simulink model "ASM_Traffic_new"  (R2024a)
settings: Solver=ode1  StartTime=SIM.tstart.v  StopTime=SIM.tend.v  FixedStep=SIM.StepSize.v  RelTol=1e-3
PostLoadFcn:
  | if any(exist('dsrtsu_mdlpostloadfcn', 'file') ~= 0), dsrtsu_mdlpostloadfcn('Execute', bdroot); end
  | try, asm_mdl_postloadfcn(bdroot, 'UpdateModel', 3600); catch, disp(lasterr); end,
InitFcn:
  | , if any(exist('rtifpga_mdlclblib', 'file') ~= 0), rtifpga_mdlclblib('Init', bdroot); end,
  | , if any(exist('dsmpb_private', 'file') ~= 0), dsmpb_private('dsmpb_mdlclblib', 'Init', bdroot); end,
undefined symbols (not defined in the file): _to_, a0b2, ASM_BrakeHydraulics_DemoSystems, ASM_VehicleDynamics_DemoSystems, b98103fe8ad365046cd0, BrakeCircuit, CPT, Crankshaft, DiscIntNeverNeededParam, dsmsi, FinalDriveAssembly, MDL, ModeSignals, Pos_BrakePedal_Maneuver, rad, RefSignals, s_to_rpm, SIM, SoftECU, Suspension, Tire, Transmission
libraries: ASM_Traffic_lib x135, simulink x100, ASM_Utils_lib x77, ASM_VehicleDynamics_lib x70, ASM_Environment_lib x22, dsmpblib x20, dsmsilib x15, MDLD_Utils_lib x10, ASM_BrakeHydraulics_lib x3
(part 2 of 63)

== system ASM_Traffic_new/ASMTools ==
  note: ---- Code Generation ----
  note: ------ Multi-Instance ------
  note: ----- Scope Handling ------
  note: ----- Signal Handling ------
  note: ------------------- Project & Experiment Handling -------------------
  note: -------------------- ModelDesk Parameter Group --------------------
  note: ------------------------------- Tire Handling -------------------------------
  ASMSignalInterface_Manager : MDLD_Utils_lib/ModelDeskPlotInterface/ASMSignalInterface_Manager
  ASM_Model_Port_Manager : ASM_Utils_lib/Miscellaneous/ASM_MODEL_PORT_MANAGER
  GenerateVEOS : ASM_Utils_lib/CodeGeneration/GenerateVEOS
  ModelDeskParaGroupOverview : ASM_Utils_lib/ModelDeskInterface/ModelDeskParaGroupOverview
  MultiInstanceOverview : ASM_Utils_lib/ModelDeskInterface/MultiInstanceOverview
  OpenExperimentModelDesk : ASM_Utils_lib/OpenExperiment/OpenExperiment  ExpDir=..\Parameterization\MOD_Traffic\Experiment_001\Experiment_001.CDE  dSProduct=ModelDesk
  ReplaceTire : ASM_Utils_lib/BlockReplacement/ReplaceVariants  editSearchPath=bdroot  popupLibBlk=<select here>  popupTargetDemo=<select here>  Demosystem=VehicleDynamics_Tire  variantLib=ASM_VehicleDynamics_DemoSystems/Tire
  ScopeHandlingGui : ASM_Utils_lib/ReplaceScopes/ScopeHandlingGui

== system ASM_Traffic_new/AnimationInterface ==
  note: Animation Interface
  In : Inport
  ANIMATION_INTERFACE : Subsystem
  Bus Selector : BusSelector  OutputSignals=Environment.Animation.Sw_AnimationInterface[0Disabled|1Enabled],Environment.Animation.ManeuverState[]
  DriverAssistance_Animation : BusSelector  OutputSignals=DomainControl.DriverAssistance.Animation  OutputAsBus=on
  Drivetrain_Animation : BusSelector  OutputSignals=Drivetrain.Animation  OutputAsBus=on
  Environment_Animation : BusSelector  OutputSignals=Environment.Animation  OutputAsBus=on
  FcnCall : Subsystem
  Fellow_Doors : Subsystem
  Fellow_Lights : Subsystem
  OpenAnimationInterfaceModel : Subsystem
      settings: OpenFcn=|
      | InterfaceModel = 'ASM_AnimationInterface';
      | 
      | try
      |     open_system(InterfaceModel);                         catch
      |     errordlg(['ERROR opening Animation interface: ',InterfaceModel,'.slx']);
      | end
      mask Display: disp('Open ASM_AnimationInterface')
  Rate Transition{,1..3} (4 alike) : RateTransition  Integrity=off  OutPortSampleTimeOpt=Inherit
  VehicleDynamics_Animation : BusSelector  OutputSignals=VehicleDynamics.Animation  OutputAsBus=on
  Vehicle_Doors : Subsystem
  Vehicle_Lights : Subsystem
  wires:
  Bus Selector/1 -> FcnCall/Enable  "<Sw_AnimationInterface[0Disabled|1Enabled]>"
  Fellow_Doors/1(Fellow_Doors) -> ANIMATION_INTERFACE/8(Fellow_Doors)
  Vehicle_Doors/1(ASM_Vehicle_Doors) -> ANIMATION_INTERFACE/7(ASM_Vehicle_Doors)
  Rate Transition2/1 -> ANIMATION_INTERFACE/4(Environment_Animation), Vehicle_Lights/2(Environment_Animation), Fellow_Doors/1(Environment_Animation), Vehicle_Doors/1(Environment_Animation), Fellow_Lights/1(Environment_Animation)
  Vehicle_Lights/1(ASM_Vehicle_Lights) -> ANIMATION_INTERFACE/5(ASM_Vehicle_Lights)
  Fellow_Lights/1(Fellow_Light) -> ANIMATION_INTERFACE/6(Fellow_Lights)
  Rate Transition3/1 -> ANIMATION_INTERFACE/3(VehicleDynamics_Animation), Vehicle_Lights/1(VehicleDynamics_Animation)
  FcnCall/1(FcnCallEvent[]) -> ANIMATION_INTERFACE/Trigger
  Bus Selector/2 -> FcnCall/1(ManeuverState[])  "<ManeuverState[]>"
  Drivetrain_Animation/1 -> Rate Transition1/1
  Rate Transition1/1 -> ANIMATION_INTERFACE/2(Drivetrain_Animation)
  Rate Transition/1 -> ANIMATION_INTERFACE/1(DriverAssistance_Animation)
  Environment_Animation/1 -> Rate Transition2/1
  DriverAssistance_Animation/1 -> Rate Transition/1
  VehicleDynamics_Animation/1 -> Rate Transition3/1
  In/1 -> VehicleDynamics_Animation/1, Environment_Animation/1, Drivetrain_Animation/1, DriverAssistance_Animation/1, Bus Selector/1

== system ASM_Traffic_new/DomainControl ==
  In : Inport
  Bus Creator : BusCreator  Inputs=3
  DriverAssistance : Subsystem
  StartSystem : Subsystem
  TorqueManager : Subsystem
  Out : Outport  VectorParamsAs1DForOutWhenUnconnected=off
  wires:
  Bus Creator/1 -> Out/1  "DomainControl"
  In/1 -> StartSystem/1(In), DriverAssistance/1(In), TorqueManager/1(In)
  DriverAssistance/1(Out) -> Bus Creator/3
  StartSystem/1(Out) -> Bus Creator/1
  TorqueManager/1(Out) -> Bus Creator/2

== system ASM_Traffic_new/Driver ==
  note: Driver
  In : Inport
  Interface_In : Subsystem
  Interface_Out : Subsystem
  Plant : Subsystem
  SignalInterface : Subsystem
  Out : Outport  VectorParamsAs1DForOutWhenUnconnected=off
  wires:
  In/1 -> Interface_In/1(In)
  Interface_In/1(Out) -> SignalInterface/1(In), Plant/1(Interface_In)
  Plant/1(Plant) -> Interface_Out/1(In)
  Interface_Out/1(Out) -> Out/1

== system ASM_Traffic_new/Drivetrain ==
  note: Drivetrain
  In : Inport
  Bus Creator1 : BusCreator  Inputs=2
  Control : Subsystem
  Interface_In : Subsystem
  Interface_Out : Subsystem
  Plant : Subsystem
  SignalInterface : Subsystem
  Out : Outport  VectorParamsAs1DForOutWhenUnconnected=off
  wires:
  Control/1(Control) -> Plant/2(Control), Bus Creator1/2
  Plant/1(Plant) -> Control/2(Plant), Bus Creator1/1
  Bus Creator1/1 -> Interface_Out/1(In)
  In/1 -> Interface_In/1(In)
  Interface_Out/1(Out) -> Out/1
  Interface_In/1(Out) -> SignalInterface/1(In), Control/1(Interface_In), Plant/1(Interface_In)

== system ASM_Traffic_new/ElectricalSystem ==
  note: Electrical System Basic
  In : Inport
  Bus Creator2 : BusCreator  Inputs=2
  Control : Subsystem
  Interface_In : Subsystem
  Interface_Out : Subsystem
  Plant : Subsystem
  SignalInterface : Subsystem
  Out : Outport  VectorParamsAs1DForOutWhenUnconnected=off
  wires:
  Bus Creator2/1 -> Interface_Out/1(In)
  Control/1(Control) -> Plant/2(Control), Bus Creator2/2
  In/1 -> Interface_In/1(In)
  Plant/1(Plant) -> Control/2(Plant), Bus Creator2/1
  Interface_Out/1(Out) -> Out/1
  Interface_In/1(Out) -> SignalInterface/1(In), Control/1(Interface_In), Plant/1(Interface_In)

== system ASM_Traffic_new/Engine ==
  note: Engine Basic
  In : Inport
  Bus Creator1 : BusCreator  Inputs=2
  Control : Subsystem
  Interface_In : Subsystem
  Interface_Out : Subsystem
  Plant : Subsystem
  SignalInterface : Subsystem
  Out : Outport  VectorParamsAs1DForOutWhenUnconnected=off
  wires:
  In/1 -> Interface_In/1(In)
  Interface_Out/1(Out) -> Out/1
  Control/1(Control) -> Plant/2(Control), Bus Creator1/2
  Interface_In/1(Out) -> SignalInterface/1(In), Control/1(Interface_In), Plant/1(Interface_In)
  Plant/1(Plant) -> Bus Creator1/1, Control/2(Plant)
  Bus Creator1/1 -> Interface_Out/1(In)

== system ASM_Traffic_new/Environment ==
  note: Environment Traffic
  In : Inport
  Bus Creator1 : BusCreator  Inputs=6
  GroundTruth : Subsystem
  Interface_In : Subsystem
  Interface_Out : Subsystem
  Maneuver : Subsystem
  ModelDesk_MC_ID_Environment : ASM_Utils_lib/ModelDeskInterface/ModelDesk_MC  Tag=ASM_MAINCOMPONENT  Editable=off  MainComponent=Environment
  Road : Subsystem
  Sensors : Subsystem
  SignalInterface : Subsystem
  Traffic : Subsystem
  Out : Outport  VectorParamsAs1DForOutWhenUnconnected=off
  wires:
  In/1 -> Interface_In/1(In)
  GroundTruth/1(Out) -> Bus Creator1/6
  Sensors/1(Out) -> Bus Creator1/5
  Interface_In/1(Out) -> Bus Creator1/1
  Bus Creator1/1 -> SignalInterface/1(In), Sensors/1(In), Traffic/1(In), Road/1(In), Maneuver/1(In), GroundTruth/1(In), Interface_Out/1(In)
  Traffic/1(Out) -> Bus Creator1/4
  Road/1(Out) -> Bus Creator1/3
  Maneuver/1(Out) -> Bus Creator1/2
  Interface_Out/1(Out) -> Out/1

== system ASM_Traffic_new/Help ==

== system ASM_Traffic_new/VehicleDynamics ==
  note: Vehicle Dynamics
  In : Inport
  Bus Creator1 : BusCreator  Inputs=2
  Control : Subsystem
  Interface_In : Subsystem
  Interface_Out : Subsystem
  Plant : Subsystem
  SignalInterface : Subsystem
  Out : Outport  VectorParamsAs1DForOutWhenUnconnected=off
  wires:
  Interface_Out/1(Out) -> Out/1
  In/1 -> Interface_In/1(In)
  Plant/1(Plant) -> Bus Creator1/1, Control/2(Plant)
  Control/1(Control) -> Plant/2(Control), Bus Creator1/2
  Interface_In/1(Out) -> SignalInterface/1(In), Control/1(Interface_In), Plant/1(Interface_In)
  Bus Creator1/1 -> Interface_Out/1(In)

== system ASM_Traffic_new/AnimationInterface/ANIMATION_INTERFACE ==
  DriverAssistance_Animation : Inport
  Drivetrain_Animation : Inport  Port=2
  VehicleDynamics_Animation : Inport  Port=3
  Environment_Animation : Inport  Port=4
  ASM_Vehicle_Lights : Inport  Port=5
  Fellow_Lights : Inport  Port=6
  ASM_Vehicle_Doors : Inport  Port=7
  Fellow_Doors : Inport  Port=8
  function : TriggerPort  TriggerType=function-call  VariantControl=Variant
  ACC_Instruments : Subsystem  Tag=Animation_ACC_Instruments  Priority=10001  Commented=on
  ASM_Vehicle : Subsystem  Tag=Animation_ASM_Vehicle  Priority=10001
  ASM_Vehicle_Instruments : Subsystem  Tag=Animation_ASM_Vehicle_Instruments  Priority=10001
  ASM_Vehicle_Occupants : Subsystem  Tag=Animation_ASM_Vehicle_Occupants  Priority=10001
  Activate_Animation : Subsystem  mask{ASMVehicle=Uncomment, ASMVehicleInstruments=Uncomment, ASMSensors=Uncomment, BoundigBoxes=Uncomment}
      mask prompts: ASMVehicle "ASM Vehicle"; ASMVehicleInstruments "ASM Vehicle Instruments"; ASMSensors "ASM Sensors"; BoundigBoxes "Bounding Boxes"
      settings: OpenFcn=|
      | subsysTag = 'Animation_Bounding_Boxes';
      | subsys = find_system(get_param(gcb,'Parent'),'SearchDepth','1','IncludeCommented','on','Tag',subsysTag);
      | if ~isempty(subsys)
      |     subsysState = get_param(subsys,'commented');
      |     if strcmp(subsysState,'off')
      |         set_param(subsys{1},'commented','on')
      |     end
      |     if strcmp(subsysState,'on')
      |         set_param(subsys{1},'commented','off')
      |     end
      | else
      |     disp(['Subsystem tagged with ''', subsysTag, ''' could not be found. The button is without action.'])
      | end
      mask TypeOptions ASMVehicle: Comment out | Uncomment
      mask Callback ASMVehicle: asm_vehicle_comment(gcb)
      mask TypeOptions ASMVehicleInstruments: Comment out | Uncomment
      mask TypeOptions ASMSensors: Comment out | Uncomment
      mask Callback ASMSensors:
      | subsys = find_system(get_param(gcb,'Parent'),'SearchDepth','1','IncludeCommented','on','Tag','ASM_Sensors');
      | if ~isempty(subsys)
      |     button_state = get_param(gcb,'ASMSensors');
      |     subsys_state = get_param(subsys,'commented');
      |     if strcmp(button_state,'Comment out') && strcmp(subsys_state,'off')
      |         set_param(subsys{1},'commented','on')
      |     end
      |     if strcmp(button_state,'Uncomment') && strcmp(subsys_state,'on')
      |         set_param(subsys{1},'commented','off')
      |     end
      | end
      mask TypeOptions BoundigBoxes: Comment out | Uncomment
      mask Display: disp('double click to\n activate/deactivate')
  Activate_Animation1 : Subsystem  mask{ASMVehicle=Uncomment, ASMVehicleInstruments=Uncomment, ASMSensors=Uncomment, BoundigBoxes=Uncomment}
      mask prompts: ASMVehicle "ASM Vehicle"; ASMVehicleInstruments "ASM Vehicle Instruments"; ASMSensors "ASM Sensors"; BoundigBoxes "Bounding Boxes"
      settings: OpenFcn=|
      | subsysTag = 'Animation_Fellows';
      | subsys = find_system(get_param(gcb,'Parent'),'SearchDepth','1','IncludeCommented','on','Tag',subsysTag);
      | if ~isempty(subsys)
      |     subsysState = get_param(subsys,'commented');
      |     if strcmp(subsysState,'off')
      |         set_param(subsys{1},'commented','on')
      |     end
      |     if strcmp(subsysState,'on')
      |         set_param(subsys{1},'commented','off')
      |     end
      | else
      |     disp(['Subsystem tagged with ''', subsysTag, ''' could not be found. The button is without action.'])
      | end
      mask TypeOptions ASMVehicle: Comment out | Uncomment
      mask Callback ASMVehicle: asm_vehicle_comment(gcb)
      mask TypeOptions ASMVehicleInstruments: Comment out | Uncomment
      mask TypeOptions ASMSensors: Comment out | Uncomment
      mask Callback ASMSensors:
      | subsys = find_system(get_param(gcb,'Parent'),'SearchDepth','1','IncludeCommented','on','Tag','ASM_Sensors');
      | if ~isempty(subsys)
      |     button_state = get_param(gcb,'ASMSensors');
      |     subsys_state = get_param(subsys,'commented');
      |     if strcmp(button_state,'Comment out') && strcmp(subsys_state,'off')
      |         set_param(subsys{1},'commented','on')
      |     end
      |     if strcmp(button_state,'Uncomment') && strcmp(subsys_state,'on')
      |         set_param(subsys{1},'commented','off')
      |     end
      | end
      mask TypeOptions BoundigBoxes: Comment out | Uncomment
      mask Display: disp('double click to\n activate/deactivate')
  Activate_Animation2 : Subsystem  mask{ASMVehicle=Uncomment, ASMVehicleInstruments=Uncomment, ASMSensors=Uncomment, BoundigBoxes=Uncomment}
      mask prompts: ASMVehicle "ASM Vehicle"; ASMVehicleInstruments "ASM Vehicle Instruments"; ASMSensors "ASM Sensors"; BoundigBoxes "Bounding Boxes"
      settings: OpenFcn=|
      | subsysTag = 'Animation_Data_Streams_Instruments';
      | subsys = find_system(get_param(gcb,'Parent'),'SearchDepth','1','IncludeCommented','on','Tag',subsysTag);
      | if ~isempty(subsys)
      |     subsysState = get_param(subsys,'commented');
      |     if strcmp(subsysState,'off')
      |         set_param(subsys{1},'commented','on')
      |     end
      |     if strcmp(subsysState,'on')
      |         set_param(subsys{1},'commented','off')
      |     end
      | else
      |     disp(['Subsystem tagged with ''', subsysTag, ''' could not be found. The button is without action.'])
      | end
      mask TypeOptions ASMVehicle: Comment out | Uncomment
      mask Callback ASMVehicle: asm_vehicle_comment(gcb)
      mask TypeOptions ASMVehicleInstruments: Comment out | Uncomment
      mask TypeOptions ASMSensors: Comment out | Uncomment
      mask Callback ASMSensors:
      | subsys = find_system(get_param(gcb,'Parent'),'SearchDepth','1','IncludeCommented','on','Tag','ASM_Sensors');
      | if ~isempty(subsys)
      |     button_state = get_param(gcb,'ASMSensors');
      |     subsys_state = get_param(subsys,'commented');
      |     if strcmp(button_state,'Comment out') && strcmp(subsys_state,'off')
      |         set_param(subsys{1},'commented','on')
      |     end
      |     if strcmp(button_state,'Uncomment') && strcmp(subsys_state,'on')
      |         set_param(subsys{1},'commented','off')
      |     end
      | end
      mask TypeOptions BoundigBoxes: Comment out | Uncomment
      mask Display: disp('double click to\n activate/deactivate')
  Activate_Animation3 : Subsystem  mask{ASMVehicle=Uncomment, ASMVehicleInstruments=Uncomment, ASMSensors=Uncomment, BoundigBoxes=Uncomment}
      mask prompts: ASMVehicle "ASM Vehicle"; ASMVehicleInstruments "ASM Vehicle Instruments"; ASMSensors "ASM Sensors"; BoundigBoxes "Bounding Boxes"
      settings: OpenFcn=|
      | subsysTag = 'Animation_Lane_Sensor';
      | subsys = find_system(get_param(gcb,'Parent'),'SearchDepth','1','IncludeCommented','on','Tag',subsysTag);
      | if ~isempty(subsys)
      |     subsysState = get_param(subsys,'commented');
      |     if strcmp(subsysState,'off')
      |         set_param(subsys{1},'commented','on')
      |     end
      |     if strcmp(subsysState,'on')
      |         set_param(subsys{1},'commented','off')
      |     end
      | else
      |     disp(['Subsystem tagged with ''', subsysTag, ''' could not be found. The button is without action.'])
      | end
      mask TypeOptions ASMVehicle: Comment out | Uncomment
      mask Callback ASMVehicle: asm_vehicle_comment(gcb)
      mask TypeOptions ASMVehicleInstruments: Comment out | Uncomment
      mask TypeOptions ASMSensors: Comment out | Uncomment
      mask Callback ASMSensors:
      | subsys = find_system(get_param(gcb,'Parent'),'SearchDepth','1','IncludeCommented','on','Tag','ASM_Sensors');
      | if ~isempty(subsys)
      |     button_state = get_param(gcb,'ASMSensors');
      |     subsys_state = get_param(subsys,'commented');
      |     if strcmp(button_state,'Comment out') && strcmp(subsys_state,'off')
      |         set_param(subsys{1},'commented','on')
      |     end
      |     if strcmp(button_state,'Uncomment') && strcmp(subsys_state,'on')
      |         set_param(subsys{1},'commented','off')
      |     end
      | end
      mask TypeOptions BoundigBoxes: Comment out | Uncomment
      mask Display: disp('double click to\n activate/deactivate')
  Activate_Animation4 : Subsystem  mask{ASMVehicle=Uncomment, ASMVehicleInstruments=Uncomment, ASMSensors=Uncomment, BoundigBoxes=Uncomment}
      mask prompts: ASMVehicle "ASM Vehicle"; ASMVehicleInstruments "ASM Vehicle Instruments"; ASMSensors "ASM Sensors"; BoundigBoxes "Bounding Boxes"
      settings: OpenFcn=|
      | subsysTag = 'Animation_Lane_Sensor_Dynamic_Instruments';
      | subsys = find_system(get_param(gcb,'Parent'),'SearchDepth','1','IncludeCommented','on','Tag',subsysTag);
      | if ~isempty(subsys)
      |     subsysState = get_param(subsys,'commented');
      |     if strcmp(subsysState,'off')
      |         set_param(subsys{1},'commented','on')
      |     end
      |     if strcmp(subsysState,'on')
      |         set_param(subsys{1},'commented','off')
      |     end
      | else
      |     disp(['Subsystem tagged with ''', subsysTag, ''' could not be found. The button is without action.'])
      | end
      mask TypeOptions ASMVehicle: Comment out | Uncomment
      mask Callback ASMVehicle: asm_vehicle_comment(gcb)
      mask TypeOptions ASMVehicleInstruments: Comment out | Uncomment
      mask TypeOptions ASMSensors: Comment out | Uncomment
      mask Callback ASMSensors:
      | subsys = find_system(get_param(gcb,'Parent'),'SearchDepth','1','IncludeCommented','on','Tag','ASM_Sensors');
      | if ~isempty(subsys)
      |     button_state = get_param(gcb,'ASMSensors');
      |     subsys_state = get_param(subsys,'commented');
      |     if strcmp(button_state,'Comment out') && strcmp(subsys_state,'off')
      |         set_param(subsys{1},'commented','on')
      |     end
      |     if strcmp(button_state,'Uncomment') && strcmp(subsys_state,'on')
      |         set_param(subsys{1},'commented','off')
      |     end
      | end
      mask TypeOptions BoundigBoxes: Comment out | Uncomment
      mask Display: disp('double click to\n activate/deactivate')
  Activate_Animation5 : Subsystem  mask{ASMVehicle=Uncomment, ASMVehicleInstruments=Uncomment, ASMSensors=Uncomment, BoundigBoxes=Uncomment}
      mask prompts: ASMVehicle "ASM Vehicle"; ASMVehicleInstruments "ASM Vehicle Instruments"; ASMSensors "ASM Sensors"; BoundigBoxes "Bounding Boxes"
      settings: OpenFcn=|
      | subsysTag = 'Animation_ACC_Instruments';
      | subsys = find_system(get_param(gcb,'Parent'),'SearchDepth','1','IncludeCommented','on','Tag',subsysTag);
      | if ~isempty(subsys)
      |     subsysState = get_param(subsys,'commented');
      |     if strcmp(subsysState,'off')
      |         set_param(subsys{1},'commented','on')
      |     end
      |     if strcmp(subsysState,'on')
      |         set_param(subsys{1},'commented','off')
      |     end
      | else
      |     disp(['Subsystem tagged with ''', subsysTag, ''' could not be found. The button is without action.'])
      | end
      mask TypeOptions ASMVehicle: Comment out | Uncomment
      mask Callback ASMVehicle: asm_vehicle_comment(gcb)
      mask TypeOptions ASMVehicleInstruments: Comment out | Uncomment
      mask TypeOptions ASMSensors: Comment out | Uncomment
      mask Callback ASMSensors:
      | subsys = find_system(get_param(gcb,'Parent'),'SearchDepth','1','IncludeCommented','on','Tag','ASM_Sensors');
      | if ~isempty(subsys)
      |     button_state = get_param(gcb,'ASMSensors');
      |     subsys_state = get_param(subsys,'commented');
      |     if strcmp(button_state,'Comment out') && strcmp(subsys_state,'off')
      |         set_param(subsys{1},'commented','on')
      |     end
      |     if strcmp(button_state,'Uncomment') && strcmp(subsys_state,'on')
      |         set_param(subsys{1},'commented','off')
      |     end
      | end
      mask TypeOptions BoundigBoxes: Comment out | Uncomment
      mask Display: disp('double click to\n activate/deactivate')
  Activate_Animation6 : Subsystem  mask{ASMVehicle=Uncomment, ASMVehicleInstruments=Uncomment, ASMSensors=Uncomment, BoundigBoxes=Uncomment}
      mask prompts: ASMVehicle "ASM Vehicle"; ASMVehicleInstruments "ASM Vehicle Instruments"; ASMSensors "ASM Sensors"; BoundigBoxes "Bounding Boxes"
      settings: OpenFcn=|
      | subsysTag = 'Animation_Sensors';
      | subsys = find_system(get_param(gcb,'Parent'),'SearchDepth','1','IncludeCommented','on','Tag',subsysTag);
      | if ~isempty(subsys)
      |     subsysState = get_param(subsys,'commented');
      |     if strcmp(subsysState,'off')
      |         set_param(subsys{1},'commented','on')
      |     end
      |     if strcmp(subsysState,'on')
      |         set_param(subsys{1},'commented','off')
      |     end
      | else
      |     disp(['Subsystem tagged with ''', subsysTag, ''' could not be found. The button is without action.'])
      | end
      mask TypeOptions ASMVehicle: Comment out | Uncomment
      mask Callback ASMVehicle: asm_vehicle_comment(gcb)
      mask TypeOptions ASMVehicleInstruments: Comment out | Uncomment
      mask TypeOptions ASMSensors: Comment out | Uncomment
      mask Callback ASMSensors:
      | subsys = find_system(get_param(gcb,'Parent'),'SearchDepth','1','IncludeCommented','on','Tag','ASM_Sensors');
      | if ~isempty(subsys)
      |     button_state = get_param(gcb,'ASMSensors');
      |     subsys_state = get_param(subsys,'commented');
      |     if strcmp(button_state,'Comment out') && strcmp(subsys_state,'off')
      |         set_param(subsys{1},'commented','on')
      |     end
      |     if strcmp(button_state,'Uncomment') && strcmp(subsys_state,'on')
      |         set_param(subsys{1},'commented','off')
      |     end
      | end
      mask TypeOptions BoundigBoxes: Comment out | Uncomment
      mask Display: disp('double click to\n activate/deactivate')
  Bounding_Boxes : Subsystem  Tag=Animation_Bounding_Boxes  Priority=10001
  Connection_Settings : Subsystem  Tag=AnimationInterface_Connection_Settings  Priority=10009  mask(Connection_Settings){CommunicationMethod=Communication Service, Sw_Mode=0, ModelStepSize=SIM.StepSize.v, NumSamples=SIM.NumSamplesAnimation.v, MaxMessageSize=65507}
      mask prompts: CommunicationMethod "Communication method"; Sw_Mode "Simulation mode [0SIL|1HIL]"; ModelStepSize "Step size of the model [s]"; NumSamples "Time steps between two sent messages []"; MaxMessageSize "Maximum message size [bytes]"
      mask help: Specifies the communication method for transferring the collected simulation data to a consuming application.
      mask TypeOptions CommunicationMethod: Ethernet TCP | Communication Service
      mask Callback CommunicationMethod:
      | CommunicationMethod = Simulink.Mask.get(gcb).getParameter('CommunicationMethod'); % Ethernet TCP; Communication Service
      | 
      |     % Get Mask Dialogs & Controls
      |     EthernetTCPDescription      = Simulink.Mask.get(gcb).getDialogControl('EthernetTCPDescription');
      |     COMServiceDescription       = Simulink.Mask.get(gcb).getDialogControl('COMServiceDescription');
      |     AdvancedSettingsContainer   = Simulink.Mask.get(gcb).getDialogControl('AdvancedSettings');
      | 
      |     % Get Ethernet TCP Parameter
      |     Sw_Mode                     = Simulink.Mask.get(gcb).getParameter('Sw_Mode'); % SIL or HIL
      | 
      |     % Get Communication Service Parameter
      |     ModelStepSize               = Simulink.Mask.get(gcb).getParameter('ModelStepSize');
      |     NumSamples                  = Simulink.Mask.get(gcb).getParameter('NumSamples');
      |     MaxMessageSize              = Simulink.Mask.get(gcb).getParameter('MaxMessageSize');
      | 
      |     % Get blocks inside the masked subsystem
      |     SwCommunicationMethod           = [gcb,'/Sw_CommunicationMethod[0TCP|1ComService]'];     % Constant block for switching the Communication Method
      |     SubSysEthernetTCP               = [gcb,'/Ethernet_TCP'];
      |     SubSysCommunicationService      = [gcb,'/Communication_Service'];
      | 
      |     if strcmp(CommunicationMethod.Value, 'Ethernet TCP')
      |         set_param(SwCommunicationMethod, 'Value','0');
      | 
      |         % Set Ethernet TCP Visibilities
      |         Sw_Mode.Visible                 = 'on';
      |         EthernetTCPDescription.Visible  = 'on';
      |         set_param(SubSysEthernetTCP,'commented','off')
      | 
      |         % Set Communication Service Visibilities
      |         AdvancedSettingsContainer.Visible   = 'off';
      |         ModelStepSize.Visible               = 'off';
      |         NumSamples.Visible                  = 'off';
      |         MaxMessageSize.Visible              = 'off';
      |         COMServiceDescription.Visible       = 'off';
      |         set_param(SubSysCommunicationService,'commented','on')
      |     elseif strcmp(CommunicationMethod.Value, 'Communication Service')
      |         set_param(SwCommunicationMethod, 'Value','1');
      | 
      |         % Set Ethernet TCP Visibilities
      |         Sw_Mode.Visible                 = 'off';
      |         EthernetTCPDescription.Visible  = 'off';
      |         set_param(SubSysEthernetTCP,'commented','on')
      | 
      |         % Set Communication Service Visibilities
      |         AdvancedSettingsContainer.Visible   = 'on';
      |         ModelStepSize.Visible               = 'on';
      |         NumSamples.Visible                  = 'on';
      |         MaxMessageSize.Visible              = 'on';
      |         COMServiceDescription.Visible       = 'on';
      |         set_param(SubSysCommunicationService,'commented','off')
      |     end
      mask Callback Sw_Mode:
      | simMode     = get_param(gcb, 'Sw_Mode');
      |     subsysSIL   = [gcb,'/Ethernet_TCP/SIL'];
      |     subsysHIL   = [gcb,'/Ethernet_TCP/HIL'];
      | 
      |     if strcmp(simMode,'0') % SIL
      |         if strcmp(get_param(subsysSIL,'commented'),'on')
      |             set_param(subsysSIL,'commented','off')
      |         end
      |         if strcmp(get_param(subsysHIL,'commented'),'off')
      |             set_param(subsysHIL,'commented','on')
      |         end
      |     elseif strcmp(simMode,'1') % HIL
      |         if strcmp(get_param(subsysHIL,'commented'),'on')
      |             set_param(subsysHIL,'commented','off')
      |         end
      |         if strcmp(get_param(subsysSIL,'commented'),'off')
      |             set_param(subsysSIL,'commented','on')
      |         end
      |     else
      |         disp(['Invalid parameter value of ''', gcb, '''. Allowed values are 0 and 1'])
      |     end
      mask TypeOptions ModelStepSize: Communication_Service/dsmsi_communication_service_BL1/ModelStepSize
      mask TypeOptions NumSamples: Communication_Service/dsmsi_communication_service_BL1/NumSamples
      mask TypeOptions MaxMessageSize: Communication_Service/dsmsi_communication_service_BL1/MaxMessageSize
      mask DialogControl EthernetTCPDescription Prompt: The Ethernet TCP connection supports the following Platforms: <br> Simulation Mode <b>SIL</b>: Simulink, VEOS <br> Simulation Mode <b>HIL</b>: SCALEXIO
      mask DialogControl COMServiceDescription Prompt: For supported platforms, please refer to the help of the "ASM_COMMUNICATION_SERVICE" block.
      mask DialogControl Settings Prompt: Settings
      mask DialogControl AdvancedSettings Prompt: Advanced settings
      mask Display: disp('Configure\n Connection Settings')
  Data_Streams_Instruments : Subsystem  Tag=Animation_Data_Streams_Instruments  Priority=10001
  Fellows : Subsystem  Tag=Animation_Fellows  Priority=10001
  Lane_Sensor : Subsystem  Tag=Animation_Lane_Sensor  Priority=10001
  Lane_Sensor_Dynamic_Instruments : Subsystem  Tag=Animation_Lane_Sensor_Dynamic_Instruments  Priority=10001  Commented=on
  Sensors : Subsystem  Tag=Animation_Sensors  Priority=10001
  Sw_Sensor_Animation[] : Constant
      settings: AttributesFormatString=1_Object3D\n2_Object2D\n3_TrafficSign\n4_LineSensor_Road_Lanes\n5_LineSensor_Road_Shape_Lines\n6_LineSensor_Road_Shape_ContObj\n7_LineSensor_Junction_Borders\n8_LineSensor_Junction_Shape_Lines\n9_LineSensor_Junction_Shape_ContObj\n10_Object3D_RadarEffects\n11_Object3D_CustomPoints
  Sw_Sensor_Selector[] : Constant
  wires:
  Environment_Animation/1 -> ASM_Vehicle_Instruments/2(Environment_Animation), Connection_Settings/1(Environment_Animation), Lane_Sensor_Dynamic_Instruments/1(Environment_Animation), Lane_Sensor/1(Environment_Animation), Fellows/1(Environment_Animation), Data_Streams_Instruments/1(Environment_Animation), Bounding_Boxes/1(Environment_Animation), Sensors/4(Environment_Animation), ASM_Vehicle_Occupants/1(Environment_Animation)
  Fellow_Doors/1 -> Fellows/3(Fellow_Doors)
  ASM_Vehicle_Doors/1 -> ASM_Vehicle/3(ASM_Vehicle_Doors)
  ASM_Vehicle_Lights/1 -> ASM_Vehicle/1(ASM_Vehicle_Lights)
  Fellow_Lights/1 -> Fellows/2(Fellow_Lights)
  Sw_Sensor_Selector[]/1 -> Sensors/2(Sw_Sensor_Selector[])
  Sw_Sensor_Animation[]/1 -> Sensors/3(Sw_Sensor_Animation[])
  Drivetrain_Animation/1 -> ASM_Vehicle_Instruments/3(Drivetrain_Animation)
  ASM_Vehicle/1(Chassis_Transformation_Matrix) -> Sensors/1(Transform_In)
  VehicleDynamics_Animation/1 -> ASM_Vehicle/2(VehicleDynamics_Animation), ASM_Vehicle_Instruments/1(VehicleDynamics_Animation)
  DriverAssistance_Animation/1 -> ACC_Instruments/1(DriverAssistance_Animation)

== system ASM_Traffic_new/AnimationInterface/FcnCall ==
  ManeuverState[] : Inport
  Enable1 : EnablePort
  Disable : Constant  Value=0  OutDataTypeStr=Inherit: Inherit via back propagation
  Enable : Constant  OutDataTypeStr=Inherit: Inherit via back propagation
  External_Samples : Subsystem  TreatAsAtomicUnit=on  SystemSampleTime=SIM.StepSize.v
      settings: AttributesFormatString=Ts=%<SystemSampleTime>
  MANEUVER_FCN_CALL_GENERATOR : ASM_Environment_lib/Environment/Maneuver/MANEUVER_FCN_CALL_GENERATOR  NumSamples=SIM.NumSamplesAnimation.v  ASMProperties=struct('Name','MANEUVER_FCN_CALL_GENERATOR','Version','3.0','Library','ASM_Environment_lib')  ASMInstanceName=maneuver_fcn_call_generator  ASMInstanceID=1
  Samples_Ext[] : Constant  OutDataTypeStr=Inherit: Inherit via back propagation
  Switch : Switch  Criteria=u2 ~= 0  SaturateOnIntegerOverflow=off  InputSameDT=off
  Switch1 : Switch  Criteria=u2 ~= 0  SaturateOnIntegerOverflow=off  InputSameDT=off
  Valid_Samples : simulink/Logic and Bit Operations/Compare To Zero  relop=>  OutDataTypeStr=boolean
  FcnCallEvent[] : Outport
  wires:
  External_Samples/1(num_Samples[]) -> Valid_Samples/1, Switch/1
  Valid_Samples/1 -> Switch1/2, Switch/2
  Switch/1 -> MANEUVER_FCN_CALL_GENERATOR/3
  Switch1/1 -> MANEUVER_FCN_CALL_GENERATOR/2
  Samples_Ext[]/1 -> Switch/3
  Enable/1 -> Switch1/1
  ManeuverState[]/1 -> MANEUVER_FCN_CALL_GENERATOR/1
  MANEUVER_FCN_CALL_GENERATOR/1 -> FcnCallEvent[]/1
  Disable/1 -> Switch1/3

== system ASM_Traffic_new/AnimationInterface/Fellow_Doors ==
  Environment_Animation : Inport
  Bus Selector1 : BusSelector  OutputSignals=UserSignals_Customized.Fellow1_DoorFL,UserSignals_Customized.Fellow2_DoorFL,UserSignals_Customized.Fellow3_DoorFL,UserSignals_Customized.Fellow4_DoorFL,UserSignals_Customized.Fellow5_DoorFL,UserSignals_Customized.Fellow6_DoorFL,UserSignals_Customized.Fellow7_DoorFL,UserSignals_Customized.Fellow8_DoorFL,UserSignals_Customized.Fellow9_DoorFL,UserSignals_Customized.Fellow10_DoorFL,UserSignals_Customized.Fellow11_DoorFL,UserSignals_Customized.Fellow12_DoorFL,UserSignals_Customized.Fellow13_DoorFL,UserSignals_Customized.Fellow14_DoorFL,UserSignals_Customized.Fellow15_DoorFL,UserSignals_Customized.Fellow16_DoorFL,UserSignals_Customized.Fellow17_DoorFL,UserSignals_Customized.Fellow18_DoorFL,UserSignals_Customized.Fellow19_DoorFL,UserSignals_Customized.Fellow20_DoorFL,UserSignals_Customized.Fellow21_DoorFL,UserSignals_Customized.Fellow22_DoorFL,UserSignals_Customized.Fellow23_DoorFL,UserSignals_Customized.Fellow24_DoorFL,UserSignals_Customized.Fellow25_DoorFL,UserSignals_Customized.Fellow26_DoorFL,UserSignals_Customized.Fellow27_DoorFL,UserSignals_Customized.Fellow28_DoorFL,UserSignals_Customized.Fellow29_DoorFL,UserSignals_Customized.Fellow30_DoorFL  OutputAsBus=on
  Bus Selector2 : BusSelector  OutputSignals=UserSignals_Customized.Fellow1_DoorFR,UserSignals_Customized.Fellow2_DoorFR,UserSignals_Customized.Fellow3_DoorFR,UserSignals_Customized.Fellow4_DoorFR,UserSignals_Customized.Fellow5_DoorFR,UserSignals_Customized.Fellow6_DoorFR,UserSignals_Customized.Fellow7_DoorFR,UserSignals_Customized.Fellow8_DoorFR,UserSignals_Customized.Fellow9_DoorFR,UserSignals_Customized.Fellow10_DoorFR,UserSignals_Customized.Fellow11_DoorFR,UserSignals_Customized.Fellow12_DoorFR,UserSignals_Customized.Fellow13_DoorFR,UserSignals_Customized.Fellow14_DoorFR,UserSignals_Customized.Fellow15_DoorFR,UserSignals_Customized.Fellow16_DoorFR,UserSignals_Customized.Fellow17_DoorFR,UserSignals_Customized.Fellow18_DoorFR,UserSignals_Customized.Fellow19_DoorFR,UserSignals_Customized.Fellow20_DoorFR,UserSignals_Customized.Fellow21_DoorFR,UserSignals_Customized.Fellow22_DoorFR,UserSignals_Customized.Fellow23_DoorFR,UserSignals_Customized.Fellow24_DoorFR,UserSignals_Customized.Fellow25_DoorFR,UserSignals_Customized.Fellow26_DoorFR,UserSignals_Customized.Fellow27_DoorFR,UserSignals_Customized.Fellow28_DoorFR,UserSignals_Customized.Fellow29_DoorFR,UserSignals_Customized.Fellow30_DoorFR  OutputAsBus=on
  Bus Selector3 : BusSelector  OutputSignals=UserSignals_Customized.Fellow1_DoorRL,UserSignals_Customized.Fellow2_DoorRL,UserSignals_Customized.Fellow3_DoorRL,UserSignals_Customized.Fellow4_DoorRL,UserSignals_Customized.Fellow5_DoorRL,UserSignals_Customized.Fellow6_DoorRL,UserSignals_Customized.Fellow7_DoorRL,UserSignals_Customized.Fellow8_DoorRL,UserSignals_Customized.Fellow9_DoorRL,UserSignals_Customized.Fellow10_DoorRL,UserSignals_Customized.Fellow11_DoorRL,UserSignals_Customized.Fellow12_DoorRL,UserSignals_Customized.Fellow13_DoorRL,UserSignals_Customized.Fellow14_DoorRL,UserSignals_Customized.Fellow15_DoorRL,UserSignals_Customized.Fellow16_DoorRL,UserSignals_Customized.Fellow17_DoorRL,UserSignals_Customized.Fellow18_DoorRL,UserSignals_Customized.Fellow19_DoorRL,UserSignals_Customized.Fellow20_DoorRL,UserSignals_Customized.Fellow21_DoorRL,UserSignals_Customized.Fellow22_DoorRL,UserSignals_Customized.Fellow23_DoorRL,UserSignals_Customized.Fellow24_DoorRL,UserSignals_Customized.Fellow25_DoorRL,UserSignals_Customized.Fellow26_DoorRL,UserSignals_Customized.Fellow27_DoorRL,UserSignals_Customized.Fellow28_DoorRL,UserSignals_Customized.Fellow29_DoorRL,UserSignals_Customized.Fellow30_DoorRL  OutputAsBus=on
  Bus Selector4 : BusSelector  OutputSignals=UserSignals_Customized.Fellow1_DoorRR,UserSignals_Customized.Fellow2_DoorRR,UserSignals_Customized.Fellow3_DoorRR,UserSignals_Customized.Fellow4_DoorRR,UserSignals_Customized.Fellow5_DoorRR,UserSignals_Customized.Fellow6_DoorRR,UserSignals_Customized.Fellow7_DoorRR,UserSignals_Customized.Fellow8_DoorRR,UserSignals_Customized.Fellow9_DoorRR,UserSignals_Customized.Fellow10_DoorRR,UserSignals_Customized.Fellow11_DoorRR,UserSignals_Customized.Fellow12_DoorRR,UserSignals_Customized.Fellow13_DoorRR,UserSignals_Customized.Fellow14_DoorRR,UserSignals_Customized.Fellow15_DoorRR,UserSignals_Customized.Fellow16_DoorRR,UserSignals_Customized.Fellow17_DoorRR,UserSignals_Customized.Fellow18_DoorRR,UserSignals_Customized.Fellow19_DoorRR,UserSignals_Customized.Fellow20_DoorRR,UserSignals_Customized.Fellow21_DoorRR,UserSignals_Customized.Fellow22_DoorRR,UserSignals_Customized.Fellow23_DoorRR,UserSignals_Customized.Fellow24_DoorRR,UserSignals_Customized.Fellow25_DoorRR,UserSignals_Customized.Fellow26_DoorRR,UserSignals_Customized.Fellow27_DoorRR,UserSignals_Customized.Fellow28_DoorRR,UserSignals_Customized.Fellow29_DoorRR,UserSignals_Customized.Fellow30_DoorRR  OutputAsBus=on
  Bus Selector5 : BusSelector  OutputSignals=UserSignals_Customized.Fellow1_Hood,UserSignals_Customized.Fellow2_Hood,UserSignals_Customized.Fellow3_Hood,UserSignals_Customized.Fellow4_Hood,UserSignals_Customized.Fellow5_Hood,UserSignals_Customized.Fellow6_Hood,UserSignals_Customized.Fellow7_Hood,UserSignals_Customized.Fellow8_Hood,UserSignals_Customized.Fellow9_Hood,UserSignals_Customized.Fellow10_Hood,UserSignals_Customized.Fellow11_Hood,UserSignals_Customized.Fellow12_Hood,UserSignals_Customized.Fellow13_Hood,UserSignals_Customized.Fellow14_Hood,UserSignals_Customized.Fellow15_Hood,UserSignals_Customized.Fellow16_Hood,UserSignals_Customized.Fellow17_Hood,UserSignals_Customized.Fellow18_Hood,UserSignals_Customized.Fellow19_Hood,UserSignals_Customized.Fellow20_Hood,UserSignals_Customized.Fellow21_Hood,UserSignals_Customized.Fellow22_Hood,UserSignals_Customized.Fellow23_Hood,UserSignals_Customized.Fellow24_Hood,UserSignals_Customized.Fellow25_Hood,UserSignals_Customized.Fellow26_Hood,UserSignals_Customized.Fellow27_Hood,UserSignals_Customized.Fellow28_Hood,UserSignals_Customized.Fellow29_Hood,UserSignals_Customized.Fellow30_Hood  OutputAsBus=on
  Bus Selector6 : BusSelector  OutputSignals=UserSignals_Customized.Fellow1_Trunk,UserSignals_Customized.Fellow2_Trunk,UserSignals_Customized.Fellow3_Trunk,UserSignals_Customized.Fellow4_Trunk,UserSignals_Customized.Fellow5_Trunk,UserSignals_Customized.Fellow6_Trunk,UserSignals_Customized.Fellow7_Trunk,UserSignals_Customized.Fellow8_Trunk,UserSignals_Customized.Fellow9_Trunk,UserSignals_Customized.Fellow10_Trunk,UserSignals_Customized.Fellow11_Trunk,UserSignals_Customized.Fellow12_Trunk,UserSignals_Customized.Fellow13_Trunk,UserSignals_Customized.Fellow14_Trunk,UserSignals_Customized.Fellow15_Trunk,UserSignals_Customized.Fellow16_Trunk,UserSignals_Customized.Fellow17_Trunk,UserSignals_Customized.Fellow18_Trunk,UserSignals_Customized.Fellow19_Trunk,UserSignals_Customized.Fellow20_Trunk,UserSignals_Customized.Fellow21_Trunk,UserSignals_Customized.Fellow22_Trunk,UserSignals_Customized.Fellow23_Trunk,UserSignals_Customized.Fellow24_Trunk,UserSignals_Customized.Fellow25_Trunk,UserSignals_Customized.Fellow26_Trunk,UserSignals_Customized.Fellow27_Trunk,UserSignals_Customized.Fellow28_Trunk,UserSignals_Customized.Fellow29_Trunk,UserSignals_Customized.Fellow30_Trunk  OutputAsBus=on
  Bus to Vector{1..6} (6 alike) : BusToVector
  Data Type Conversion{1..6} (6 alike) : DataTypeConversion  OutDataTypeStr=double  SaturateOnIntegerOverflow=off  RndMeth=Floor
  Multiport Switch : MultiPortSwitch  Inputs=2  OutMin=30  OutMax=30  OutDataTypeStr=double  SaturateOnIntegerOverflow=off
  Multiport Switch{1..5} (5 alike) : MultiPortSwitch  Inputs=2  SaturateOnIntegerOverflow=off  InputSameDT=off
  Mux : Mux  Inputs=6
  Saturation : Saturate  UpperLimit=1  LowerLimit=0
  Select_Signals : Subsystem
  Fellow_Doors : Outport  VectorParamsAs1DForOutWhenUnconnected=off
  wires:
  Saturation/1 -> Fellow_Doors/1
  Environment_Animation/1 -> Select_Signals/1(Fellow_Doors), Bus Selector1/1, Bus Selector3/1, Bus Selector4/1, Bus Selector5/1, Bus Selector6/1, Bus Selector2/1
  Mux/1 -> Saturation/1
  Multiport Switch/1 -> Mux/1
  Multiport Switch1/1 -> Mux/2
  Multiport Switch2/1 -> Mux/3
  Multiport Switch3/1 -> Mux/4
  Multiport Switch5/1 -> Mux/6
  Multiport Switch4/1 -> Mux/5
  Select_Signals/7(SW_Trunk[Open0_1Closed]) -> Multiport Switch5/3
  Select_Signals/6(SW_Hood[Open0_1Closed]) -> Multiport Switch4/3
  Select_Signals/5(SW_DoorRR[Open0_1Closed]) -> Multiport Switch3/3
  Select_Signals/4(SW_DoorRL[Open0_1Closed]) -> Multiport Switch2/3
  Select_Signals/3(SW_DoorFR[Open0_1Closed]) -> Multiport Switch1/3
  Data Type Conversion2/1 -> Multiport Switch1/2
  Data Type Conversion3/1 -> Multiport Switch2/2
  Data Type Conversion4/1 -> Multiport Switch3/2
  Bus Selector6/1 -> Bus to Vector6/1
  Data Type Conversion6/1 -> Multiport Switch5/2
  Bus to Vector6/1 -> Data Type Conversion6/1
  Bus Selector5/1 -> Bus to Vector5/1
  Data Type Conversion5/1 -> Multiport Switch4/2
  Bus to Vector5/1 -> Data Type Conversion5/1
  Bus Selector4/1 -> Bus to Vector4/1
  Bus to Vector4/1 -> Data Type Conversion4/1
  Bus Selector3/1 -> Bus to Vector3/1
  Bus to Vector3/1 -> Data Type Conversion3/1
  Bus Selector2/1 -> Bus to Vector2/1
  Bus to Vector2/1 -> Data Type Conversion2/1
  Data Type Conversion1/1 -> Multiport Switch/2
  Bus to Vector1/1 -> Data Type Conversion1/1
  Bus Selector1/1 -> Bus to Vector1/1
  Select_Signals/2(SW_DoorFL[Open0_1Closed]) -> Multiport Switch/3
  Select_Signals/1(SW_ManualControl_Doors[1Scheduler|2Manual]) -> Multiport Switch/1, Multiport Switch1/1, Multiport Switch2/1, Multiport Switch3/1, Multiport Switch4/1, Multiport Switch5/1

== system ASM_Traffic_new/AnimationInterface/Fellow_Lights ==
  Environment_Animation : Inport
  Bus Selector : BusSelector  OutputSignals=Fellow1_TurnLights,Fellow2_TurnLights,Fellow3_TurnLights,Fellow4_TurnLights,Fellow5_TurnLights,Fellow6_TurnLights,Fellow7_TurnLights,Fellow8_TurnLights,Fellow9_TurnLights,Fellow10_TurnLights,Fellow11_TurnLights,Fellow12_TurnLights,Fellow13_TurnLights,Fellow14_TurnLights,Fellow15_TurnLights,Fellow16_TurnLights,Fellow17_TurnLights,Fellow18_TurnLights,Fellow19_TurnLights,Fellow20_TurnLights,Fellow21_TurnLights,Fellow22_TurnLights,Fellow23_TurnLights,Fellow24_TurnLights,Fellow25_TurnLights,Fellow26_TurnLights,Fellow27_TurnLights,Fellow28_TurnLights,Fellow29_TurnLights,Fellow30_TurnLights  OutputAsBus=on
  Bus Selector2 : BusSelector  OutputSignals=a_Fellows[m|s2],Settings,UserSignals_Customized
  Bus to Vector3 : BusToVector
  Coding : Subsystem
  Compare_Both : simulink/Logic and Bit Operations/Compare To Constant  relop===  const=3  OutDataTypeStr=boolean
  Compare_Turnlight_L : simulink/Logic and Bit Operations/Compare To Constant  relop===  const=1  OutDataTypeStr=boolean
  Compare_Turnlight_R : simulink/Logic and Bit Operations/Compare To Constant  relop===  const=2  OutDataTypeStr=boolean
  Gain : Gain  Gain=-1
  Multiport Switch : MultiPortSwitch  Inputs=2  SaturateOnIntegerOverflow=off  InputSameDT=off
  Multiport Switch4 : MultiPortSwitch  Inputs=2  SaturateOnIntegerOverflow=off  InputSameDT=off
  Mux : Mux  Inputs=3
  OR : Logic  Operator=OR  IconShape=distinctive  AllPortsSameDT=off  OutDataTypeStr=boolean
  OR1 : Logic  Operator=OR  IconShape=distinctive  AllPortsSameDT=off  OutDataTypeStr=boolean
  Relay : Relay  OnSwitchValue=1.3  OffSwitchValue=1.2  OutDataTypeStr=boolean
  Select_Signals : Subsystem
  TurnLights[0|1|2|3] : DataTypeConversion  OutDataTypeStr=uint32  SaturateOnIntegerOverflow=off  RndMeth=Floor
  Fellow_Light : Outport  VectorParamsAs1DForOutWhenUnconnected=off
  wires:
  Gain/1 -> Relay/1
  Bus Selector2/2 -> Select_Signals/1(Fellow_VehicleLights)  "<Settings>"
  Environment_Animation/1 -> Bus Selector2/1
  Select_Signals/3(SW_TurnLight[0Off|1Left|2Right|3Both]) -> Multiport Switch4/3
  Select_Signals/2(SW_BrakeLight[0Off|1On]) -> Multiport Switch/3
  Select_Signals/1(SW_ManualControl_Lights[1Scheduler|2Manual]) -> Multiport Switch/1, Multiport Switch4/1
  Bus to Vector3/1 -> TurnLights[0|1|2|3]/1
  Mux/1 -> Coding/1(FellowLights)
  Multiport Switch4/1 -> Compare_Both/1, Compare_Turnlight_R/1, Compare_Turnlight_L/1
  OR1/1 -> Mux/3
  OR/1 -> Mux/2
  Compare_Both/1 -> OR/2, OR1/2
  Multiport Switch/1 -> Mux/1
  Compare_Turnlight_R/1 -> OR1/1
  Compare_Turnlight_L/1 -> OR/1
  Relay/1 -> Multiport Switch/2
  TurnLights[0|1|2|3]/1 -> Multiport Switch4/2
  Coding/1(Out) -> Fellow_Light/1
  Bus Selector2/1 -> Gain/1  "<a_Fellows[m|s2]>"
  Bus Selector2/3 -> Bus Selector/1  "<UserSignals_Customized>"
  Bus Selector/1 -> Bus to Vector3/1

== system ASM_Traffic_new/AnimationInterface/OpenAnimationInterfaceModel ==

== system ASM_Traffic_new/AnimationInterface/Vehicle_Doors ==
  Environment_Animation : Inport
  Bus Selector : BusSelector  OutputSignals=Mnv_DoorFL[],Mnv_DoorFR[],Mnv_DoorRL[],Mnv_DoorRR[],Mnv_Hood[],Mnv_Trunk[]  OutputAsBus=on
  Bus Selector7 : BusSelector  OutputSignals=Sw_ManualControl_Doors[1Maneuver|2Manual]
  Bus Selector8 : BusSelector  OutputSignals=Sw_DoorFL[0Closed_1Open],Sw_DoorFR[0Closed_1Open],Sw_DoorRL[0Closed_1Open],Sw_DoorRR[0Closed_1Open],Sw_Hood[0Closed_1Open],Sw_Trunk[0Closed_1Open]  OutputAsBus=on
  Bus to Vector : BusToVector
  Bus to Vector7 : BusToVector
  Data Type Conversion : DataTypeConversion  OutDataTypeStr=double  SaturateOnIntegerOverflow=off  RndMeth=Floor
  Data Type Conversion7 : DataTypeConversion  OutDataTypeStr=uint32  SaturateOnIntegerOverflow=off  RndMeth=Floor
  Data Type Conversion8 : DataTypeConversion  OutDataTypeStr=double  SaturateOnIntegerOverflow=off  RndMeth=Floor
  Multiport Switch6 : MultiPortSwitch  Inputs=2  OutMin=30  OutMax=30  OutDataTypeStr=double  SaturateOnIntegerOverflow=off
  Saturation : Saturate  UpperLimit=1  LowerLimit=0
  ASM_Vehicle_Doors : Outport  VectorParamsAs1DForOutWhenUnconnected=off
  wires:
  Saturation/1 -> ASM_Vehicle_Doors/1
  Data Type Conversion7/1 -> Multiport Switch6/1
  Bus Selector7/1 -> Data Type Conversion7/1  "<Sw_ManualControl_Doors[1Maneuver|2Manual]>"
  Data Type Conversion8/1 -> Multiport Switch6/3
  Multiport Switch6/1 -> Saturation/1
  Bus to Vector7/1 -> Data Type Conversion8/1
  Bus to Vector/1 -> Data Type Conversion/1
  Bus Selector8/1 -> Bus to Vector7/1
  Data Type Conversion/1 -> Multiport Switch6/2
  Environment_Animation/1 -> Bus Selector/1, Bus Selector7/1, Bus Selector8/1
  Bus Selector/1 -> Bus to Vector/1
